simulink model "MMC_21_Level_Rectifier"  (R2023b)
settings: Solver=FixedStepAuto  StartTime=0.0  StopTime=0.5  RelTol=1e-3
libraries: spsSeriesRLCBranchLib x71, spsVoltageMeasurementLib x69, spsUniversalBridgeLib x60, spsCurrentMeasurementLib x8, slpidlib x7, spsRMSLib x3, spsACVoltageSourceLib x3, spsMeanLib x2, simulink x1, spsTHDLib x1, spspowerguiLib x1
(part 3 of 4)

== system MMC_21_Level_Rectifier/三电平级联混合MMC/Subsystem1/Subsystem/混合三电平子模块5 ==
  DRV : Inport
  C0 : spsSeriesRLCBranchLib/Series RLC Branch  LConnTagsString=__new0  RConnTagsString=__new0  BranchType=C  Resistance=0.1  Inductance=0  SetiL0=off  InitialCurrent=0  Capacitance=2e-3  Setx0=on  InitialVoltage=2200  Measurements=None
  C1 : spsSeriesRLCBranchLib/Series RLC Branch  LConnTagsString=__new0  RConnTagsString=__new0  BranchType=C  Resistance=0.1  Inductance=0  SetiL0=off  InitialCurrent=0  Capacitance=2e-3  Setx0=on  InitialVoltage=2200  Measurements=None
  Demux3 : Demux  Outputs=2
  Mux : Mux  Inputs=2
  Universal Bridge1 : spsUniversalBridgeLib/Universal Bridge  Arms=1  SnubberResistance=1e6  SnubberCapacitance=inf  Device=IGBT / Diodes  Ron=1e-3  Lon=0  ForwardVoltages="[  1  1  ]"  ForwardVoltage=0  GTOparameters=[ 10e-6 , 20e-6 ]  IGBTparameters=[ 1e-6 , 2e-6 ]  Measurements=None  Measurements_2=None  converterType=Rectifier
  Universal Bridge2 : spsUniversalBridgeLib/Universal Bridge  Arms=1  SnubberResistance=1e6  SnubberCapacitance=inf  Device=IGBT / Diodes  Ron=1e-3  Lon=0  ForwardVoltages="[  1  1  ]"  ForwardVoltage=0  GTOparameters=[ 10e-6 , 20e-6 ]  IGBTparameters=[ 1e-6 , 2e-6 ]  Measurements=None  Measurements_2=None  converterType=Rectifier
  Vm1 : spsVoltageMeasurementLib/Voltage Measurement  PhasorSimulation=off  OutputType=Complex  PSBequivalent=0
  Vm3 : spsVoltageMeasurementLib/Voltage Measurement  PhasorSimulation=off  OutputType=Complex  PSBequivalent=0
  A : PMIOPort  Side=Left
  B : PMIOPort  Port=2  Side=Left
  Udc : Outport
  wires:
  Mux/1 -> Udc/1
  DRV/1 -> Demux3/1
  Demux3/2 -> Universal Bridge2/1
  Vm1/1 -> Mux/1
  Vm3/1 -> Mux/2
  Demux3/1 -> Universal Bridge1/1
  connections:
  Vm1/LConn2 -- C0/RConn1 -- Universal Bridge1/RConn2 -- Universal Bridge2/LConn1
  Universal Bridge1/LConn1 -- A/RConn1
  Vm3/LConn1 -- C1/LConn1 -- Universal Bridge2/RConn1
  Vm1/LConn1 -- Universal Bridge1/RConn1 -- C0/LConn1
  Universal Bridge2/RConn2 -- C1/RConn1 -- B/RConn1 -- Vm3/LConn2

== system MMC_21_Level_Rectifier/三电平级联混合MMC/Subsystem1/Subsystem1/混合三电平子模块1 ==
  DRV : Inport
  C0 : spsSeriesRLCBranchLib/Series RLC Branch  LConnTagsString=__new0  RConnTagsString=__new0  BranchType=C  Resistance=0.1  Inductance=0  SetiL0=off  InitialCurrent=0  Capacitance=2e-3  Setx0=on  InitialVoltage=2200  Measurements=None
  C1 : spsSeriesRLCBranchLib/Series RLC Branch  LConnTagsString=__new0  RConnTagsString=__new0  BranchType=C  Resistance=0.1  Inductance=0  SetiL0=off  InitialCurrent=0  Capacitance=2e-3  Setx0=on  InitialVoltage=2200  Measurements=None
  Demux3 : Demux  Outputs=2
  Mux : Mux  Inputs=2
  Universal Bridge1 : spsUniversalBridgeLib/Universal Bridge  Arms=1  SnubberResistance=1e6  SnubberCapacitance=inf  Device=IGBT / Diodes  Ron=1e-3  Lon=0  ForwardVoltages="[  1  1  ]"  ForwardVoltage=0  GTOparameters=[ 10e-6 , 20e-6 ]  IGBTparameters=[ 1e-6 , 2e-6 ]  Measurements=None  Measurements_2=None  converterType=Rectifier
  Universal Bridge2 : spsUniversalBridgeLib/Universal Bridge  Arms=1  SnubberResistance=1e6  SnubberCapacitance=inf  Device=IGBT / Diodes  Ron=1e-3  Lon=0  ForwardVoltages="[  1  1  ]"  ForwardVoltage=0  GTOparameters=[ 10e-6 , 20e-6 ]  IGBTparameters=[ 1e-6 , 2e-6 ]  Measurements=None  Measurements_2=None  converterType=Rectifier
  Vm1 : spsVoltageMeasurementLib/Voltage Measurement  PhasorSimulation=off  OutputType=Complex  PSBequivalent=0
  Vm3 : spsVoltageMeasurementLib/Voltage Measurement  PhasorSimulation=off  OutputType=Complex  PSBequivalent=0
  A : PMIOPort  Side=Left
  B : PMIOPort  Port=2  Side=Left
  Udc : Outport
  wires:
  Demux3/1 -> Universal Bridge1/1
  Vm3/1 -> Mux/2
  Vm1/1 -> Mux/1
  Demux3/2 -> Universal Bridge2/1
  DRV/1 -> Demux3/1
  Mux/1 -> Udc/1
  connections:
  Vm3/LConn2 -- B/RConn1 -- C1/RConn1 -- Universal Bridge2/RConn2
  C0/LConn1 -- Universal Bridge1/RConn1 -- Vm1/LConn1
  Universal Bridge2/RConn1 -- C1/LConn1 -- Vm3/LConn1
  Universal Bridge1/LConn1 -- A/RConn1
  Universal Bridge2/LConn1 -- Universal Bridge1/RConn2 -- C0/RConn1 -- Vm1/LConn2

== system MMC_21_Level_Rectifier/三电平级联混合MMC/Subsystem1/Subsystem1/混合三电平子模块2 ==
  DRV : Inport
  C0 : spsSeriesRLCBranchLib/Series RLC Branch  LConnTagsString=__new0  RConnTagsString=__new0  BranchType=C  Resistance=0.1  Inductance=0  SetiL0=off  InitialCurrent=0  Capacitance=2e-3  Setx0=on  InitialVoltage=2200  Measurements=None
  C1 : spsSeriesRLCBranchLib/Series RLC Branch  LConnTagsString=__new0  RConnTagsString=__new0  BranchType=C  Resistance=0.1  Inductance=0  SetiL0=off  InitialCurrent=0  Capacitance=2e-3  Setx0=on  InitialVoltage=2200  Measurements=None
  Demux3 : Demux  Outputs=2
  Mux : Mux  Inputs=2
  Universal Bridge1 : spsUniversalBridgeLib/Universal Bridge  Arms=1  SnubberResistance=1e6  SnubberCapacitance=inf  Device=IGBT / Diodes  Ron=1e-3  Lon=0  ForwardVoltages="[  1  1  ]"  ForwardVoltage=0  GTOparameters=[ 10e-6 , 20e-6 ]  IGBTparameters=[ 1e-6 , 2e-6 ]  Measurements=None  Measurements_2=None  converterType=Rectifier
  Universal Bridge2 : spsUniversalBridgeLib/Universal Bridge  Arms=1  SnubberResistance=1e6  SnubberCapacitance=inf  Device=IGBT / Diodes  Ron=1e-3  Lon=0  ForwardVoltages="[  1  1  ]"  ForwardVoltage=0  GTOparameters=[ 10e-6 , 20e-6 ]  IGBTparameters=[ 1e-6 , 2e-6 ]  Measurements=None  Measurements_2=None  converterType=Rectifier
  Vm1 : spsVoltageMeasurementLib/Voltage Measurement  PhasorSimulation=off  OutputType=Complex  PSBequivalent=0
  Vm3 : spsVoltageMeasurementLib/Voltage Measurement  PhasorSimulation=off  OutputType=Complex  PSBequivalent=0
  A : PMIOPort  Side=Left
  B : PMIOPort  Port=2  Side=Left
  Udc : Outport
  wires:
  Mux/1 -> Udc/1
  DRV/1 -> Demux3/1
  Demux3/2 -> Universal Bridge2/1
  Vm1/1 -> Mux/1
  Vm3/1 -> Mux/2
  Demux3/1 -> Universal Bridge1/1
  connections:
  Vm1/LConn2 -- C0/RConn1 -- Universal Bridge1/RConn2 -- Universal Bridge2/LConn1
  Universal Bridge1/LConn1 -- A/RConn1
  Vm3/LConn1 -- C1/LConn1 -- Universal Bridge2/RConn1
  Vm1/LConn1 -- Universal Bridge1/RConn1 -- C0/LConn1
  Universal Bridge2/RConn2 -- C1/RConn1 -- B/RConn1 -- Vm3/LConn2

== system MMC_21_Level_Rectifier/三电平级联混合MMC/Subsystem1/Subsystem1/混合三电平子模块3 ==
  DRV : Inport
  C0 : spsSeriesRLCBranchLib/Series RLC Branch  LConnTagsString=__new0  RConnTagsString=__new0  BranchType=C  Resistance=0.1  Inductance=0  SetiL0=off  InitialCurrent=0  Capacitance=2e-3  Setx0=on  InitialVoltage=2200  Measurements=None
  C1 : spsSeriesRLCBranchLib/Series RLC Branch  LConnTagsString=__new0  RConnTagsString=__new0  BranchType=C  Resistance=0.1  Inductance=0  SetiL0=off  InitialCurrent=0  Capacitance=2e-3  Setx0=on  InitialVoltage=2200  Measurements=None
  Demux3 : Demux  Outputs=2
  Mux : Mux  Inputs=2
  Universal Bridge1 : spsUniversalBridgeLib/Universal Bridge  Arms=1  SnubberResistance=1e6  SnubberCapacitance=inf  Device=IGBT / Diodes  Ron=1e-3  Lon=0  ForwardVoltages="[  1  1  ]"  ForwardVoltage=0  GTOparameters=[ 10e-6 , 20e-6 ]  IGBTparameters=[ 1e-6 , 2e-6 ]  Measurements=None  Measurements_2=None  converterType=Rectifier
  Universal Bridge2 : spsUniversalBridgeLib/Universal Bridge  Arms=1  SnubberResistance=1e6  SnubberCapacitance=inf  Device=IGBT / Diodes  Ron=1e-3  Lon=0  ForwardVoltages="[  1  1  ]"  ForwardVoltage=0  GTOparameters=[ 10e-6 , 20e-6 ]  IGBTparameters=[ 1e-6 , 2e-6 ]  Measurements=None  Measurements_2=None  converterType=Rectifier
  Vm1 : spsVoltageMeasurementLib/Voltage Measurement  PhasorSimulation=off  OutputType=Complex  PSBequivalent=0
  Vm3 : spsVoltageMeasurementLib/Voltage Measurement  PhasorSimulation=off  OutputType=Complex  PSBequivalent=0
  A : PMIOPort  Side=Left
  B : PMIOPort  Port=2  Side=Left
  Udc : Outport
  wires:
  Demux3/1 -> Universal Bridge1/1
  Vm3/1 -> Mux/2
  Vm1/1 -> Mux/1
  Demux3/2 -> Universal Bridge2/1
  DRV/1 -> Demux3/1
  Mux/1 -> Udc/1
  connections:
  Vm3/LConn2 -- B/RConn1 -- C1/RConn1 -- Universal Bridge2/RConn2
  C0/LConn1 -- Universal Bridge1/RConn1 -- Vm1/LConn1
  Universal Bridge2/RConn1 -- C1/LConn1 -- Vm3/LConn1
  Universal Bridge1/LConn1 -- A/RConn1
  Universal Bridge2/LConn1 -- Universal Bridge1/RConn2 -- C0/RConn1 -- Vm1/LConn2

== system MMC_21_Level_Rectifier/三电平级联混合MMC/Subsystem1/Subsystem1/混合三电平子模块4 ==
  DRV : Inport
  C0 : spsSeriesRLCBranchLib/Series RLC Branch  LConnTagsString=__new0  RConnTagsString=__new0  BranchType=C  Resistance=0.1  Inductance=0  SetiL0=off  InitialCurrent=0  Capacitance=2e-3  Setx0=on  InitialVoltage=2200  Measurements=None
  C1 : spsSeriesRLCBranchLib/Series RLC Branch  LConnTagsString=__new0  RConnTagsString=__new0  BranchType=C  Resistance=0.1  Inductance=0  SetiL0=off  InitialCurrent=0  Capacitance=2e-3  Setx0=on  InitialVoltage=2200  Measurements=None
  Demux3 : Demux  Outputs=2
  Mux : Mux  Inputs=2
  Universal Bridge1 : spsUniversalBridgeLib/Universal Bridge  Arms=1  SnubberResistance=1e6  SnubberCapacitance=inf  Device=IGBT / Diodes  Ron=1e-3  Lon=0  ForwardVoltages="[  1  1  ]"  ForwardVoltage=0  GTOparameters=[ 10e-6 , 20e-6 ]  IGBTparameters=[ 1e-6 , 2e-6 ]  Measurements=None  Measurements_2=None  converterType=Rectifier
  Universal Bridge2 : spsUniversalBridgeLib/Universal Bridge  Arms=1  SnubberResistance=1e6  SnubberCapacitance=inf  Device=IGBT / Diodes  Ron=1e-3  Lon=0  ForwardVoltages="[  1  1  ]"  ForwardVoltage=0  GTOparameters=[ 10e-6 , 20e-6 ]  IGBTparameters=[ 1e-6 , 2e-6 ]  Measurements=None  Measurements_2=None  converterType=Rectifier
  Vm1 : spsVoltageMeasurementLib/Voltage Measurement  PhasorSimulation=off  OutputType=Complex  PSBequivalent=0
  Vm3 : spsVoltageMeasurementLib/Voltage Measurement  PhasorSimulation=off  OutputType=Complex  PSBequivalent=0
  A : PMIOPort  Side=Left
  B : PMIOPort  Port=2  Side=Left
  Udc : Outport
  wires:
  Mux/1 -> Udc/1
  DRV/1 -> Demux3/1
  Demux3/2 -> Universal Bridge2/1
  Vm1/1 -> Mux/1
  Vm3/1 -> Mux/2
  Demux3/1 -> Universal Bridge1/1
  connections:
  Vm1/LConn2 -- C0/RConn1 -- Universal Bridge1/RConn2 -- Universal Bridge2/LConn1
  Universal Bridge1/LConn1 -- A/RConn1
  Vm3/LConn1 -- C1/LConn1 -- Universal Bridge2/RConn1
  Vm1/LConn1 -- Universal Bridge1/RConn1 -- C0/LConn1
  Universal Bridge2/RConn2 -- C1/RConn1 -- B/RConn1 -- Vm3/LConn2

== system MMC_21_Level_Rectifier/三电平级联混合MMC/Subsystem1/Subsystem1/混合三电平子模块5 ==
  DRV : Inport
  C0 : spsSeriesRLCBranchLib/Series RLC Branch  LConnTagsString=__new0  RConnTagsString=__new0  BranchType=C  Resistance=0.1  Inductance=0  SetiL0=off  InitialCurrent=0  Capacitance=2e-3  Setx0=on  InitialVoltage=2200  Measurements=None
  C1 : spsSeriesRLCBranchLib/Series RLC Branch  LConnTagsString=__new0  RConnTagsString=__new0  BranchType=C  Resistance=0.1  Inductance=0  SetiL0=off  InitialCurrent=0  Capacitance=2e-3  Setx0=on  InitialVoltage=2200  Measurements=None
  Demux3 : Demux  Outputs=2
  Mux : Mux  Inputs=2
  Universal Bridge1 : spsUniversalBridgeLib/Universal Bridge  Arms=1  SnubberResistance=1e6  SnubberCapacitance=inf  Device=IGBT / Diodes  Ron=1e-3  Lon=0  ForwardVoltages="[  1  1  ]"  ForwardVoltage=0  GTOparameters=[ 10e-6 , 20e-6 ]  IGBTparameters=[ 1e-6 , 2e-6 ]  Measurements=None  Measurements_2=None  converterType=Rectifier
  Universal Bridge2 : spsUniversalBridgeLib/Universal Bridge  Arms=1  SnubberResistance=1e6  SnubberCapacitance=inf  Device=IGBT / Diodes  Ron=1e-3  Lon=0  ForwardVoltages="[  1  1  ]"  ForwardVoltage=0  GTOparameters=[ 10e-6 , 20e-6 ]  IGBTparameters=[ 1e-6 , 2e-6 ]  Measurements=None  Measurements_2=None  converterType=Rectifier
  Vm1 : spsVoltageMeasurementLib/Voltage Measurement  PhasorSimulation=off  OutputType=Complex  PSBequivalent=0
  Vm3 : spsVoltageMeasurementLib/Voltage Measurement  PhasorSimulation=off  OutputType=Complex  PSBequivalent=0
  A : PMIOPort  Side=Left
  B : PMIOPort  Port=2  Side=Left
  Udc : Outport
  wires:
  Demux3/1 -> Universal Bridge1/1
  Vm3/1 -> Mux/2
  Vm1/1 -> Mux/1
  Demux3/2 -> Universal Bridge2/1
  DRV/1 -> Demux3/1
  Mux/1 -> Udc/1
  connections:
  Vm3/LConn2 -- B/RConn1 -- C1/RConn1 -- Universal Bridge2/RConn2
  C0/LConn1 -- Universal Bridge1/RConn1 -- Vm1/LConn1
  Universal Bridge2/RConn1 -- C1/LConn1 -- Vm3/LConn1
  Universal Bridge1/LConn1 -- A/RConn1
  Universal Bridge2/LConn1 -- Universal Bridge1/RConn2 -- C0/RConn1 -- Vm1/LConn2

== system MMC_21_Level_Rectifier/三电平级联混合MMC/Subsystem2/Subsystem/混合三电平子模块1 ==
  DRV : Inport
  C0 : spsSeriesRLCBranchLib/Series RLC Branch  LConnTagsString=__new0  RConnTagsString=__new0  BranchType=C  Resistance=0.1  Inductance=0  SetiL0=off  InitialCurrent=0  Capacitance=2e-3  Setx0=on  InitialVoltage=2200  Measurements=None
  C1 : spsSeriesRLCBranchLib/Series RLC Branch  LConnTagsString=__new0  RConnTagsString=__new0  BranchType=C  Resistance=0.1  Inductance=0  SetiL0=off  InitialCurrent=0  Capacitance=2e-3  Setx0=on  InitialVoltage=2200  Measurements=None
  Demux3 : Demux  Outputs=2
  Mux : Mux  Inputs=2
  Universal Bridge1 : spsUniversalBridgeLib/Universal Bridge  Arms=1  SnubberResistance=1e6  SnubberCapacitance=inf  Device=IGBT / Diodes  Ron=1e-3  Lon=0  ForwardVoltages="[  1  1  ]"  ForwardVoltage=0  GTOparameters=[ 10e-6 , 20e-6 ]  IGBTparameters=[ 1e-6 , 2e-6 ]  Measurements=None  Measurements_2=None  converterType=Rectifier
  Universal Bridge2 : spsUniversalBridgeLib/Universal Bridge  Arms=1  SnubberResistance=1e6  SnubberCapacitance=inf  Device=IGBT / Diodes  Ron=1e-3  Lon=0  ForwardVoltages="[  1  1  ]"  ForwardVoltage=0  GTOparameters=[ 10e-6 , 20e-6 ]  IGBTparameters=[ 1e-6 , 2e-6 ]  Measurements=None  Measurements_2=None  converterType=Rectifier
  Vm1 : spsVoltageMeasurementLib/Voltage Measurement  PhasorSimulation=off  OutputType=Complex  PSBequivalent=0
  Vm3 : spsVoltageMeasurementLib/Voltage Measurement  PhasorSimulation=off  OutputType=Complex  PSBequivalent=0
  A : PMIOPort  Side=Left
  B : PMIOPort  Port=2  Side=Left
  Udc : Outport
  wires:
  Demux3/1 -> Universal Bridge1/1
  Vm3/1 -> Mux/2
  Vm1/1 -> Mux/1
  Demux3/2 -> Universal Bridge2/1
  DRV/1 -> Demux3/1
  Mux/1 -> Udc/1
  connections:
  C1/RConn1 -- Universal Bridge2/RConn2 -- Vm3/LConn2 -- B/RConn1
  C0/LConn1 -- Universal Bridge1/RConn1 -- Vm1/LConn1
  C1/LConn1 -- Vm3/LConn1 -- Universal Bridge2/RConn1
  Universal Bridge1/LConn1 -- A/RConn1
  C0/RConn1 -- Universal Bridge2/LConn1 -- Vm1/LConn2 -- Universal Bridge1/RConn2

== system MMC_21_Level_Rectifier/三电平级联混合MMC/Subsystem2/Subsystem/混合三电平子模块2 ==
  DRV : Inport
  C0 : spsSeriesRLCBranchLib/Series RLC Branch  LConnTagsString=__new0  RConnTagsString=__new0  BranchType=C  Resistance=0.1  Inductance=0  SetiL0=off  InitialCurrent=0  Capacitance=2e-3  Setx0=on  InitialVoltage=2200  Measurements=None
  C1 : spsSeriesRLCBranchLib/Series RLC Branch  LConnTagsString=__new0  RConnTagsString=__new0  BranchType=C  Resistance=0.1  Inductance=0  SetiL0=off  InitialCurrent=0  Capacitance=2e-3  Setx0=on  InitialVoltage=2200  Measurements=None
  Demux3 : Demux  Outputs=2
  Mux : Mux  Inputs=2
  Universal Bridge1 : spsUniversalBridgeLib/Universal Bridge  Arms=1  SnubberResistance=1e6  SnubberCapacitance=inf  Device=IGBT / Diodes  Ron=1e-3  Lon=0  ForwardVoltages="[  1  1  ]"  ForwardVoltage=0  GTOparameters=[ 10e-6 , 20e-6 ]  IGBTparameters=[ 1e-6 , 2e-6 ]  Measurements=None  Measurements_2=None  converterType=Rectifier
  Universal Bridge2 : spsUniversalBridgeLib/Universal Bridge  Arms=1  SnubberResistance=1e6  SnubberCapacitance=inf  Device=IGBT / Diodes  Ron=1e-3  Lon=0  ForwardVoltages="[  1  1  ]"  ForwardVoltage=0  GTOparameters=[ 10e-6 , 20e-6 ]  IGBTparameters=[ 1e-6 , 2e-6 ]  Measurements=None  Measurements_2=None  converterType=Rectifier
  Vm1 : spsVoltageMeasurementLib/Voltage Measurement  PhasorSimulation=off  OutputType=Complex  PSBequivalent=0
  Vm3 : spsVoltageMeasurementLib/Voltage Measurement  PhasorSimulation=off  OutputType=Complex  PSBequivalent=0
  A : PMIOPort  Side=Left
  B : PMIOPort  Port=2  Side=Left
  Udc : Outport
  wires:
  Mux/1 -> Udc/1
  DRV/1 -> Demux3/1
  Demux3/2 -> Universal Bridge2/1
  Vm1/1 -> Mux/1
  Vm3/1 -> Mux/2
  Demux3/1 -> Universal Bridge1/1
  connections:
  Vm1/LConn2 -- C0/RConn1 -- Universal Bridge1/RConn2 -- Universal Bridge2/LConn1
  Universal Bridge1/LConn1 -- A/RConn1
  Vm3/LConn1 -- C1/LConn1 -- Universal Bridge2/RConn1
  Vm1/LConn1 -- Universal Bridge1/RConn1 -- C0/LConn1
  Universal Bridge2/RConn2 -- C1/RConn1 -- B/RConn1 -- Vm3/LConn2

== system MMC_21_Level_Rectifier/三电平级联混合MMC/Subsystem2/Subsystem/混合三电平子模块3 ==
  DRV : Inport
  C0 : spsSeriesRLCBranchLib/Series RLC Branch  LConnTagsString=__new0  RConnTagsString=__new0  BranchType=C  Resistance=0.1  Inductance=0  SetiL0=off  InitialCurrent=0  Capacitance=2e-3  Setx0=on  InitialVoltage=2200  Measurements=None
  C1 : spsSeriesRLCBranchLib/Series RLC Branch  LConnTagsString=__new0  RConnTagsString=__new0  BranchType=C  Resistance=0.1  Inductance=0  SetiL0=off  InitialCurrent=0  Capacitance=2e-3  Setx0=on  InitialVoltage=2200  Measurements=None
  Demux3 : Demux  Outputs=2
  Mux : Mux  Inputs=2
  Universal Bridge1 : spsUniversalBridgeLib/Universal Bridge  Arms=1  SnubberResistance=1e6  SnubberCapacitance=inf  Device=IGBT / Diodes  Ron=1e-3  Lon=0  ForwardVoltages="[  1  1  ]"  ForwardVoltage=0  GTOparameters=[ 10e-6 , 20e-6 ]  IGBTparameters=[ 1e-6 , 2e-6 ]  Measurements=None  Measurements_2=None  converterType=Rectifier
  Universal Bridge2 : spsUniversalBridgeLib/Universal Bridge  Arms=1  SnubberResistance=1e6  SnubberCapacitance=inf  Device=IGBT / Diodes  Ron=1e-3  Lon=0  ForwardVoltages="[  1  1  ]"  ForwardVoltage=0  GTOparameters=[ 10e-6 , 20e-6 ]  IGBTparameters=[ 1e-6 , 2e-6 ]  Measurements=None  Measurements_2=None  converterType=Rectifier
  Vm1 : spsVoltageMeasurementLib/Voltage Measurement  PhasorSimulation=off  OutputType=Complex  PSBequivalent=0
  Vm3 : spsVoltageMeasurementLib/Voltage Measurement  PhasorSimulation=off  OutputType=Complex  PSBequivalent=0
  A : PMIOPort  Side=Left
  B : PMIOPort  Port=2  Side=Left
  Udc : Outport
  wires:
  Demux3/1 -> Universal Bridge1/1
  Vm3/1 -> Mux/2
  Vm1/1 -> Mux/1
  Demux3/2 -> Universal Bridge2/1
  DRV/1 -> Demux3/1
  Mux/1 -> Udc/1
  connections:
  Vm3/LConn2 -- B/RConn1 -- C1/RConn1 -- Universal Bridge2/RConn2
  C0/LConn1 -- Universal Bridge1/RConn1 -- Vm1/LConn1
  Universal Bridge2/RConn1 -- C1/LConn1 -- Vm3/LConn1
  Universal Bridge1/LConn1 -- A/RConn1
  Universal Bridge2/LConn1 -- Universal Bridge1/RConn2 -- C0/RConn1 -- Vm1/LConn2

== system MMC_21_Level_Rectifier/三电平级联混合MMC/Subsystem2/Subsystem/混合三电平子模块4 ==
  DRV : Inport
  C0 : spsSeriesRLCBranchLib/Series RLC Branch  LConnTagsString=__new0  RConnTagsString=__new0  BranchType=C  Resistance=0.1  Inductance=0  SetiL0=off  InitialCurrent=0  Capacitance=2e-3  Setx0=on  InitialVoltage=2200  Measurements=None
  C1 : spsSeriesRLCBranchLib/Series RLC Branch  LConnTagsString=__new0  RConnTagsString=__new0  BranchType=C  Resistance=0.1  Inductance=0  SetiL0=off  InitialCurrent=0  Capacitance=2e-3  Setx0=on  InitialVoltage=2200  Measurements=None
  Demux3 : Demux  Outputs=2
  Mux : Mux  Inputs=2
  Universal Bridge1 : spsUniversalBridgeLib/Universal Bridge  Arms=1  SnubberResistance=1e6  SnubberCapacitance=inf  Device=IGBT / Diodes  Ron=1e-3  Lon=0  ForwardVoltages="[  1  1  ]"  ForwardVoltage=0  GTOparameters=[ 10e-6 , 20e-6 ]  IGBTparameters=[ 1e-6 , 2e-6 ]  Measurements=None  Measurements_2=None  converterType=Rectifier
  Universal Bridge2 : spsUniversalBridgeLib/Universal Bridge  Arms=1  SnubberResistance=1e6  SnubberCapacitance=inf  Device=IGBT / Diodes  Ron=1e-3  Lon=0  ForwardVoltages="[  1  1  ]"  ForwardVoltage=0  GTOparameters=[ 10e-6 , 20e-6 ]  IGBTparameters=[ 1e-6 , 2e-6 ]  Measurements=None  Measurements_2=None  converterType=Rectifier
  Vm1 : spsVoltageMeasurementLib/Voltage Measurement  PhasorSimulation=off  OutputType=Complex  PSBequivalent=0
  Vm3 : spsVoltageMeasurementLib/Voltage Measurement  PhasorSimulation=off  OutputType=Complex  PSBequivalent=0
  A : PMIOPort  Side=Left
  B : PMIOPort  Port=2  Side=Left
  Udc : Outport
  wires:
  Mux/1 -> Udc/1
  DRV/1 -> Demux3/1
  Demux3/2 -> Universal Bridge2/1
  Vm1/1 -> Mux/1
  Vm3/1 -> Mux/2
  Demux3/1 -> Universal Bridge1/1
  connections:
  Vm1/LConn2 -- C0/RConn1 -- Universal Bridge1/RConn2 -- Universal Bridge2/LConn1
  Universal Bridge1/LConn1 -- A/RConn1
  Vm3/LConn1 -- C1/LConn1 -- Universal Bridge2/RConn1
  Vm1/LConn1 -- Universal Bridge1/RConn1 -- C0/LConn1
  Universal Bridge2/RConn2 -- C1/RConn1 -- B/RConn1 -- Vm3/LConn2

== system MMC_21_Level_Rectifier/三电平级联混合MMC/Subsystem2/Subsystem/混合三电平子模块5 ==
  DRV : Inport
  C0 : spsSeriesRLCBranchLib/Series RLC Branch  LConnTagsString=__new0  RConnTagsString=__new0  BranchType=C  Resistance=0.1  Inductance=0  SetiL0=off  InitialCurrent=0  Capacitance=2e-3  Setx0=on  InitialVoltage=2200  Measurements=None
  C1 : spsSeriesRLCBranchLib/Series RLC Branch  LConnTagsString=__new0  RConnTagsString=__new0  BranchType=C  Resistance=0.1  Inductance=0  SetiL0=off  InitialCurrent=0  Capacitance=2e-3  Setx0=on  InitialVoltage=2200  Measurements=None
  Demux3 : Demux  Outputs=2
  Mux : Mux  Inputs=2
  Universal Bridge1 : spsUniversalBridgeLib/Universal Bridge  Arms=1  SnubberResistance=1e6  SnubberCapacitance=inf  Device=IGBT / Diodes  Ron=1e-3  Lon=0  ForwardVoltages="[  1  1  ]"  ForwardVoltage=0  GTOparameters=[ 10e-6 , 20e-6 ]  IGBTparameters=[ 1e-6 , 2e-6 ]  Measurements=None  Measurements_2=None  converterType=Rectifier
  Universal Bridge2 : spsUniversalBridgeLib/Universal Bridge  Arms=1  SnubberResistance=1e6  SnubberCapacitance=inf  Device=IGBT / Diodes  Ron=1e-3  Lon=0  ForwardVoltages="[  1  1  ]"  ForwardVoltage=0  GTOparameters=[ 10e-6 , 20e-6 ]  IGBTparameters=[ 1e-6 , 2e-6 ]  Measurements=None  Measurements_2=None  converterType=Rectifier
  Vm1 : spsVoltageMeasurementLib/Voltage Measurement  PhasorSimulation=off  OutputType=Complex  PSBequivalent=0
  Vm3 : spsVoltageMeasurementLib/Voltage Measurement  PhasorSimulation=off  OutputType=Complex  PSBequivalent=0
  A : PMIOPort  Side=Left
  B : PMIOPort  Port=2  Side=Left
  Udc : Outport
  wires:
  Demux3/1 -> Universal Bridge1/1
  Vm3/1 -> Mux/2
  Vm1/1 -> Mux/1
  Demux3/2 -> Universal Bridge2/1
  DRV/1 -> Demux3/1
  Mux/1 -> Udc/1
  connections:
  Vm3/LConn2 -- B/RConn1 -- C1/RConn1 -- Universal Bridge2/RConn2
  C0/LConn1 -- Universal Bridge1/RConn1 -- Vm1/LConn1
  Universal Bridge2/RConn1 -- C1/LConn1 -- Vm3/LConn1
  Universal Bridge1/LConn1 -- A/RConn1
  Universal Bridge2/LConn1 -- Universal Bridge1/RConn2 -- C0/RConn1 -- Vm1/LConn2

== system MMC_21_Level_Rectifier/三电平级联混合MMC/Subsystem2/Subsystem1/混合三电平子模块1 ==
  DRV : Inport
  C0 : spsSeriesRLCBranchLib/Series RLC Branch  LConnTagsString=__new0  RConnTagsString=__new0  BranchType=C  Resistance=0.1  Inductance=0  SetiL0=off  InitialCurrent=0  Capacitance=2e-3  Setx0=on  InitialVoltage=2200  Measurements=None
  C1 : spsSeriesRLCBranchLib/Series RLC Branch  LConnTagsString=__new0  RConnTagsString=__new0  BranchType=C  Resistance=0.1  Inductance=0  SetiL0=off  InitialCurrent=0  Capacitance=2e-3  Setx0=on  InitialVoltage=2200  Measurements=None
  Demux3 : Demux  Outputs=2
  Mux : Mux  Inputs=2
  Universal Bridge1 : spsUniversalBridgeLib/Universal Bridge  Arms=1  SnubberResistance=1e6  SnubberCapacitance=inf  Device=IGBT / Diodes  Ron=1e-3  Lon=0  ForwardVoltages="[  1  1  ]"  ForwardVoltage=0  GTOparameters=[ 10e-6 , 20e-6 ]  IGBTparameters=[ 1e-6 , 2e-6 ]  Measurements=None  Measurements_2=None  converterType=Rectifier
  Universal Bridge2 : spsUniversalBridgeLib/Universal Bridge  Arms=1  SnubberResistance=1e6  SnubberCapacitance=inf  Device=IGBT / Diodes  Ron=1e-3  Lon=0  ForwardVoltages="[  1  1  ]"  ForwardVoltage=0  GTOparameters=[ 10e-6 , 20e-6 ]  IGBTparameters=[ 1e-6 , 2e-6 ]  Measurements=None  Measurements_2=None  converterType=Rectifier
  Vm1 : spsVoltageMeasurementLib/Voltage Measurement  PhasorSimulation=off  OutputType=Complex  PSBequivalent=0
  Vm3 : spsVoltageMeasurementLib/Voltage Measurement  PhasorSimulation=off  OutputType=Complex  PSBequivalent=0
  A : PMIOPort  Side=Left
  B : PMIOPort  Port=2  Side=Left
  Udc : Outport
  wires:
  Mux/1 -> Udc/1
  DRV/1 -> Demux3/1
  Demux3/2 -> Universal Bridge2/1
  Vm1/1 -> Mux/1
  Vm3/1 -> Mux/2
  Demux3/1 -> Universal Bridge1/1
  connections:
  Vm1/LConn2 -- C0/RConn1 -- Universal Bridge1/RConn2 -- Universal Bridge2/LConn1
  Universal Bridge1/LConn1 -- A/RConn1
  Vm3/LConn1 -- C1/LConn1 -- Universal Bridge2/RConn1
  Vm1/LConn1 -- Universal Bridge1/RConn1 -- C0/LConn1
  Universal Bridge2/RConn2 -- C1/RConn1 -- B/RConn1 -- Vm3/LConn2

== system MMC_21_Level_Rectifier/三电平级联混合MMC/Subsystem2/Subsystem1/混合三电平子模块2 ==
  DRV : Inport
  C0 : spsSeriesRLCBranchLib/Series RLC Branch  LConnTagsString=__new0  RConnTagsString=__new0  BranchType=C  Resistance=0.1  Inductance=0  SetiL0=off  InitialCurrent=0  Capacitance=2e-3  Setx0=on  InitialVoltage=2200  Measurements=None
  C1 : spsSeriesRLCBranchLib/Series RLC Branch  LConnTagsString=__new0  RConnTagsString=__new0  BranchType=C  Resistance=0.1  Inductance=0  SetiL0=off  InitialCurrent=0  Capacitance=2e-3  Setx0=on  InitialVoltage=2200  Measurements=None
  Demux3 : Demux  Outputs=2
  Mux : Mux  Inputs=2
  Universal Bridge1 : spsUniversalBridgeLib/Universal Bridge  Arms=1  SnubberResistance=1e6  SnubberCapacitance=inf  Device=IGBT / Diodes  Ron=1e-3  Lon=0  ForwardVoltages="[  1  1  ]"  ForwardVoltage=0  GTOparameters=[ 10e-6 , 20e-6 ]  IGBTparameters=[ 1e-6 , 2e-6 ]  Measurements=None  Measurements_2=None  converterType=Rectifier
  Universal Bridge2 : spsUniversalBridgeLib/Universal Bridge  Arms=1  SnubberResistance=1e6  SnubberCapacitance=inf  Device=IGBT / Diodes  Ron=1e-3  Lon=0  ForwardVoltages="[  1  1  ]"  ForwardVoltage=0  GTOparameters=[ 10e-6 , 20e-6 ]  IGBTparameters=[ 1e-6 , 2e-6 ]  Measurements=None  Measurements_2=None  converterType=Rectifier
  Vm1 : spsVoltageMeasurementLib/Voltage Measurement  PhasorSimulation=off  OutputType=Complex  PSBequivalent=0
  Vm3 : spsVoltageMeasurementLib/Voltage Measurement  PhasorSimulation=off  OutputType=Complex  PSBequivalent=0
  A : PMIOPort  Side=Left
  B : PMIOPort  Port=2  Side=Left
  Udc : Outport
  wires:
  Demux3/1 -> Universal Bridge1/1
  Vm3/1 -> Mux/2
  Vm1/1 -> Mux/1
  Demux3/2 -> Universal Bridge2/1
  DRV/1 -> Demux3/1
  Mux/1 -> Udc/1
  connections:
  Vm3/LConn2 -- B/RConn1 -- C1/RConn1 -- Universal Bridge2/RConn2
  C0/LConn1 -- Universal Bridge1/RConn1 -- Vm1/LConn1
  Universal Bridge2/RConn1 -- C1/LConn1 -- Vm3/LConn1
  Universal Bridge1/LConn1 -- A/RConn1
  Universal Bridge2/LConn1 -- Universal Bridge1/RConn2 -- C0/RConn1 -- Vm1/LConn2

== system MMC_21_Level_Rectifier/三电平级联混合MMC/Subsystem2/Subsystem1/混合三电平子模块3 ==
  DRV : Inport
  C0 : spsSeriesRLCBranchLib/Series RLC Branch  LConnTagsString=__new0  RConnTagsString=__new0  BranchType=C  Resistance=0.1  Inductance=0  SetiL0=off  InitialCurrent=0  Capacitance=2e-3  Setx0=on  InitialVoltage=2200  Measurements=None
  C1 : spsSeriesRLCBranchLib/Series RLC Branch  LConnTagsString=__new0  RConnTagsString=__new0  BranchType=C  Resistance=0.1  Inductance=0  SetiL0=off  InitialCurrent=0  Capacitance=2e-3  Setx0=on  InitialVoltage=2200  Measurements=None
  Demux3 : Demux  Outputs=2
  Mux : Mux  Inputs=2
  Universal Bridge1 : spsUniversalBridgeLib/Universal Bridge  Arms=1  SnubberResistance=1e6  SnubberCapacitance=inf  Device=IGBT / Diodes  Ron=1e-3  Lon=0  ForwardVoltages="[  1  1  ]"  ForwardVoltage=0  GTOparameters=[ 10e-6 , 20e-6 ]  IGBTparameters=[ 1e-6 , 2e-6 ]  Measurements=None  Measurements_2=None  converterType=Rectifier
  Universal Bridge2 : spsUniversalBridgeLib/Universal Bridge  Arms=1  SnubberResistance=1e6  SnubberCapacitance=inf  Device=IGBT / Diodes  Ron=1e-3  Lon=0  ForwardVoltages="[  1  1  ]"  ForwardVoltage=0  GTOparameters=[ 10e-6 , 20e-6 ]  IGBTparameters=[ 1e-6 , 2e-6 ]  Measurements=None  Measurements_2=None  converterType=Rectifier
  Vm1 : spsVoltageMeasurementLib/Voltage Measurement  PhasorSimulation=off  OutputType=Complex  PSBequivalent=0
  Vm3 : spsVoltageMeasurementLib/Voltage Measurement  PhasorSimulation=off  OutputType=Complex  PSBequivalent=0
  A : PMIOPort  Side=Left
  B : PMIOPort  Port=2  Side=Left
  Udc : Outport
  wires:
  Mux/1 -> Udc/1
  DRV/1 -> Demux3/1
  Demux3/2 -> Universal Bridge2/1
  Vm1/1 -> Mux/1
  Vm3/1 -> Mux/2
  Demux3/1 -> Universal Bridge1/1
  connections:
  Vm1/LConn2 -- C0/RConn1 -- Universal Bridge1/RConn2 -- Universal Bridge2/LConn1
  Universal Bridge1/LConn1 -- A/RConn1
  Vm3/LConn1 -- C1/LConn1 -- Universal Bridge2/RConn1
  Vm1/LConn1 -- Universal Bridge1/RConn1 -- C0/LConn1
  Universal Bridge2/RConn2 -- C1/RConn1 -- B/RConn1 -- Vm3/LConn2

== system MMC_21_Level_Rectifier/三电平级联混合MMC/Subsystem2/Subsystem1/混合三电平子模块4 ==
  DRV : Inport
  C0 : spsSeriesRLCBranchLib/Series RLC Branch  LConnTagsString=__new0  RConnTagsString=__new0  BranchType=C  Resistance=0.1  Inductance=0  SetiL0=off  InitialCurrent=0  Capacitance=2e-3  Setx0=on  InitialVoltage=2200  Measurements=None
  C1 : spsSeriesRLCBranchLib/Series RLC Branch  LConnTagsString=__new0  RConnTagsString=__new0  BranchType=C  Resistance=0.1  Inductance=0  SetiL0=off  InitialCurrent=0  Capacitance=2e-3  Setx0=on  InitialVoltage=2200  Measurements=None
  Demux3 : Demux  Outputs=2
  Mux : Mux  Inputs=2
  Universal Bridge1 : spsUniversalBridgeLib/Universal Bridge  Arms=1  SnubberResistance=1e6  SnubberCapacitance=inf  Device=IGBT / Diodes  Ron=1e-3  Lon=0  ForwardVoltages="[  1  1  ]"  ForwardVoltage=0  GTOparameters=[ 10e-6 , 20e-6 ]  IGBTparameters=[ 1e-6 , 2e-6 ]  Measurements=None  Measurements_2=None  converterType=Rectifier
  Universal Bridge2 : spsUniversalBridgeLib/Universal Bridge  Arms=1  SnubberResistance=1e6  SnubberCapacitance=inf  Device=IGBT / Diodes  Ron=1e-3  Lon=0  ForwardVoltages="[  1  1  ]"  ForwardVoltage=0  GTOparameters=[ 10e-6 , 20e-6 ]  IGBTparameters=[ 1e-6 , 2e-6 ]  Measurements=None  Measurements_2=None  converterType=Rectifier
  Vm1 : spsVoltageMeasurementLib/Voltage Measurement  PhasorSimulation=off  OutputType=Complex  PSBequivalent=0
  Vm3 : spsVoltageMeasurementLib/Voltage Measurement  PhasorSimulation=off  OutputType=Complex  PSBequivalent=0
  A : PMIOPort  Side=Left
  B : PMIOPort  Port=2  Side=Left
  Udc : Outport
  wires:
  Demux3/1 -> Universal Bridge1/1
  Vm3/1 -> Mux/2
  Vm1/1 -> Mux/1
  Demux3/2 -> Universal Bridge2/1
  DRV/1 -> Demux3/1
  Mux/1 -> Udc/1
  connections:
  Vm3/LConn2 -- B/RConn1 -- C1/RConn1 -- Universal Bridge2/RConn2
  C0/LConn1 -- Universal Bridge1/RConn1 -- Vm1/LConn1
  Universal Bridge2/RConn1 -- C1/LConn1 -- Vm3/LConn1
  Universal Bridge1/LConn1 -- A/RConn1
  Universal Bridge2/LConn1 -- Universal Bridge1/RConn2 -- C0/RConn1 -- Vm1/LConn2

== system MMC_21_Level_Rectifier/三电平级联混合MMC/Subsystem2/Subsystem1/混合三电平子模块5 ==
  DRV : Inport
  C0 : spsSeriesRLCBranchLib/Series RLC Branch  LConnTagsString=__new0  RConnTagsString=__new0  BranchType=C  Resistance=0.1  Inductance=0  SetiL0=off  InitialCurrent=0  Capacitance=2e-3  Setx0=on  InitialVoltage=2200  Measurements=None
  C1 : spsSeriesRLCBranchLib/Series RLC Branch  LConnTagsString=__new0  RConnTagsString=__new0  BranchType=C  Resistance=0.1  Inductance=0  SetiL0=off  InitialCurrent=0  Capacitance=2e-3  Setx0=on  InitialVoltage=2200  Measurements=None
  Demux3 : Demux  Outputs=2
  Mux : Mux  Inputs=2
  Universal Bridge1 : spsUniversalBridgeLib/Universal Bridge  Arms=1  SnubberResistance=1e6  SnubberCapacitance=inf  Device=IGBT / Diodes  Ron=1e-3  Lon=0  ForwardVoltages="[  1  1  ]"  ForwardVoltage=0  GTOparameters=[ 10e-6 , 20e-6 ]  IGBTparameters=[ 1e-6 , 2e-6 ]  Measurements=None  Measurements_2=None  converterType=Rectifier
  Universal Bridge2 : spsUniversalBridgeLib/Universal Bridge  Arms=1  SnubberResistance=1e6  SnubberCapacitance=inf  Device=IGBT / Diodes  Ron=1e-3  Lon=0  ForwardVoltages="[  1  1  ]"  ForwardVoltage=0  GTOparameters=[ 10e-6 , 20e-6 ]  IGBTparameters=[ 1e-6 , 2e-6 ]  Measurements=None  Measurements_2=None  converterType=Rectifier
  Vm1 : spsVoltageMeasurementLib/Voltage Measurement  PhasorSimulation=off  OutputType=Complex  PSBequivalent=0
  Vm3 : spsVoltageMeasurementLib/Voltage Measurement  PhasorSimulation=off  OutputType=Complex  PSBequivalent=0
  A : PMIOPort  Side=Left
  B : PMIOPort  Port=2  Side=Left
  Udc : Outport
  wires:
  Mux/1 -> Udc/1
  DRV/1 -> Demux3/1
  Demux3/2 -> Universal Bridge2/1
  Vm1/1 -> Mux/1
  Vm3/1 -> Mux/2
  Demux3/1 -> Universal Bridge1/1
  connections:
  Vm1/LConn2 -- C0/RConn1 -- Universal Bridge1/RConn2 -- Universal Bridge2/LConn1
  Universal Bridge1/LConn1 -- A/RConn1
  Vm3/LConn1 -- C1/LConn1 -- Universal Bridge2/RConn1
  Vm1/LConn1 -- Universal Bridge1/RConn1 -- C0/LConn1
  Universal Bridge2/RConn2 -- C1/RConn1 -- B/RConn1 -- Vm3/LConn2

== system MMC_21_Level_Rectifier/三电平级联混合MMC/Subsystem3/Subsystem/混合三电平子模块1 ==
  DRV : Inport
  C0 : spsSeriesRLCBranchLib/Series RLC Branch  LConnTagsString=__new0  RConnTagsString=__new0  BranchType=C  Resistance=0.1  Inductance=0  SetiL0=off  InitialCurrent=0  Capacitance=2e-3  Setx0=on  InitialVoltage=2200  Measurements=None
  C1 : spsSeriesRLCBranchLib/Series RLC Branch  LConnTagsString=__new0  RConnTagsString=__new0  BranchType=C  Resistance=0.1  Inductance=0  SetiL0=off  InitialCurrent=0  Capacitance=2e-3  Setx0=on  InitialVoltage=2200  Measurements=None
  Demux3 : Demux  Outputs=2
  Mux : Mux  Inputs=2
  Universal Bridge1 : spsUniversalBridgeLib/Universal Bridge  Arms=1  SnubberResistance=1e6  SnubberCapacitance=inf  Device=IGBT / Diodes  Ron=1e-3  Lon=0  ForwardVoltages="[  1  1  ]"  ForwardVoltage=0  GTOparameters=[ 10e-6 , 20e-6 ]  IGBTparameters=[ 1e-6 , 2e-6 ]  Measurements=None  Measurements_2=None  converterType=Rectifier
  Universal Bridge2 : spsUniversalBridgeLib/Universal Bridge  Arms=1  SnubberResistance=1e6  SnubberCapacitance=inf  Device=IGBT / Diodes  Ron=1e-3  Lon=0  ForwardVoltages="[  1  1  ]"  ForwardVoltage=0  GTOparameters=[ 10e-6 , 20e-6 ]  IGBTparameters=[ 1e-6 , 2e-6 ]  Measurements=None  Measurements_2=None  converterType=Rectifier
  Vm1 : spsVoltageMeasurementLib/Voltage Measurement  PhasorSimulation=off  OutputType=Complex  PSBequivalent=0
  Vm3 : spsVoltageMeasurementLib/Voltage Measurement  PhasorSimulation=off  OutputType=Complex  PSBequivalent=0
  A : PMIOPort  Side=Left
  B : PMIOPort  Port=2  Side=Left
  Udc : Outport
  wires:
  Demux3/1 -> Universal Bridge1/1
  Vm3/1 -> Mux/2
  Vm1/1 -> Mux/1
  Demux3/2 -> Universal Bridge2/1
  DRV/1 -> Demux3/1
  Mux/1 -> Udc/1
  connections:
  Vm3/LConn2 -- B/RConn1 -- C1/RConn1 -- Universal Bridge2/RConn2
  C0/LConn1 -- Universal Bridge1/RConn1 -- Vm1/LConn1
  Universal Bridge2/RConn1 -- C1/LConn1 -- Vm3/LConn1
  Universal Bridge1/LConn1 -- A/RConn1
  Universal Bridge2/LConn1 -- Universal Bridge1/RConn2 -- C0/RConn1 -- Vm1/LConn2

== system MMC_21_Level_Rectifier/三电平级联混合MMC/Subsystem3/Subsystem/混合三电平子模块2 ==
  DRV : Inport
  C0 : spsSeriesRLCBranchLib/Series RLC Branch  LConnTagsString=__new0  RConnTagsString=__new0  BranchType=C  Resistance=0.1  Inductance=0  SetiL0=off  InitialCurrent=0  Capacitance=2e-3  Setx0=on  InitialVoltage=2200  Measurements=None
  C1 : spsSeriesRLCBranchLib/Series RLC Branch  LConnTagsString=__new0  RConnTagsString=__new0  BranchType=C  Resistance=0.1  Inductance=0  SetiL0=off  InitialCurrent=0  Capacitance=2e-3  Setx0=on  InitialVoltage=2200  Measurements=None
  Demux3 : Demux  Outputs=2
  Mux : Mux  Inputs=2
  Universal Bridge1 : spsUniversalBridgeLib/Universal Bridge  Arms=1  SnubberResistance=1e6  SnubberCapacitance=inf  Device=IGBT / Diodes  Ron=1e-3  Lon=0  ForwardVoltages="[  1  1  ]"  ForwardVoltage=0  GTOparameters=[ 10e-6 , 20e-6 ]  IGBTparameters=[ 1e-6 , 2e-6 ]  Measurements=None  Measurements_2=None  converterType=Rectifier
  Universal Bridge2 : spsUniversalBridgeLib/Universal Bridge  Arms=1  SnubberResistance=1e6  SnubberCapacitance=inf  Device=IGBT / Diodes  Ron=1e-3  Lon=0  ForwardVoltages="[  1  1  ]"  ForwardVoltage=0  GTOparameters=[ 10e-6 , 20e-6 ]  IGBTparameters=[ 1e-6 , 2e-6 ]  Measurements=None  Measurements_2=None  converterType=Rectifier
  Vm1 : spsVoltageMeasurementLib/Voltage Measurement  PhasorSimulation=off  OutputType=Complex  PSBequivalent=0
  Vm3 : spsVoltageMeasurementLib/Voltage Measurement  PhasorSimulation=off  OutputType=Complex  PSBequivalent=0
  A : PMIOPort  Side=Left
  B : PMIOPort  Port=2  Side=Left
  Udc : Outport
  wires:
  Mux/1 -> Udc/1
  DRV/1 -> Demux3/1
  Demux3/2 -> Universal Bridge2/1
  Vm1/1 -> Mux/1
  Vm3/1 -> Mux/2
  Demux3/1 -> Universal Bridge1/1
  connections:
  Vm1/LConn2 -- C0/RConn1 -- Universal Bridge1/RConn2 -- Universal Bridge2/LConn1
  Universal Bridge1/LConn1 -- A/RConn1
  Vm3/LConn1 -- C1/LConn1 -- Universal Bridge2/RConn1
  Vm1/LConn1 -- Universal Bridge1/RConn1 -- C0/LConn1
  Universal Bridge2/RConn2 -- C1/RConn1 -- B/RConn1 -- Vm3/LConn2

== system MMC_21_Level_Rectifier/三电平级联混合MMC/Subsystem3/Subsystem/混合三电平子模块3 ==
  DRV : Inport
  C0 : spsSeriesRLCBranchLib/Series RLC Branch  LConnTagsString=__new0  RConnTagsString=__new0  BranchType=C  Resistance=0.1  Inductance=0  SetiL0=off  InitialCurrent=0  Capacitance=2e-3  Setx0=on  InitialVoltage=2200  Measurements=None
  C1 : spsSeriesRLCBranchLib/Series RLC Branch  LConnTagsString=__new0  RConnTagsString=__new0  BranchType=C  Resistance=0.1  Inductance=0  SetiL0=off  InitialCurrent=0  Capacitance=2e-3  Setx0=on  InitialVoltage=2200  Measurements=None
  Demux3 : Demux  Outputs=2
  Mux : Mux  Inputs=2
  Universal Bridge1 : spsUniversalBridgeLib/Universal Bridge  Arms=1  SnubberResistance=1e6  SnubberCapacitance=inf  Device=IGBT / Diodes  Ron=1e-3  Lon=0  ForwardVoltages="[  1  1  ]"  ForwardVoltage=0  GTOparameters=[ 10e-6 , 20e-6 ]  IGBTparameters=[ 1e-6 , 2e-6 ]  Measurements=None  Measurements_2=None  converterType=Rectifier
  Universal Bridge2 : spsUniversalBridgeLib/Universal Bridge  Arms=1  SnubberResistance=1e6  SnubberCapacitance=inf  Device=IGBT / Diodes  Ron=1e-3  Lon=0  ForwardVoltages="[  1  1  ]"  ForwardVoltage=0  GTOparameters=[ 10e-6 , 20e-6 ]  IGBTparameters=[ 1e-6 , 2e-6 ]  Measurements=None  Measurements_2=None  converterType=Rectifier
  Vm1 : spsVoltageMeasurementLib/Voltage Measurement  PhasorSimulation=off  OutputType=Complex  PSBequivalent=0
  Vm3 : spsVoltageMeasurementLib/Voltage Measurement  PhasorSimulation=off  OutputType=Complex  PSBequivalent=0
  A : PMIOPort  Side=Left
  B : PMIOPort  Port=2  Side=Left
  Udc : Outport
  wires:
  Demux3/1 -> Universal Bridge1/1
  Vm3/1 -> Mux/2
  Vm1/1 -> Mux/1
  Demux3/2 -> Universal Bridge2/1
  DRV/1 -> Demux3/1
  Mux/1 -> Udc/1
  connections:
  Vm3/LConn2 -- B/RConn1 -- C1/RConn1 -- Universal Bridge2/RConn2
  C0/LConn1 -- Universal Bridge1/RConn1 -- Vm1/LConn1
  Universal Bridge2/RConn1 -- C1/LConn1 -- Vm3/LConn1
  Universal Bridge1/LConn1 -- A/RConn1
  Universal Bridge2/LConn1 -- Universal Bridge1/RConn2 -- C0/RConn1 -- Vm1/LConn2

== system MMC_21_Level_Rectifier/三电平级联混合MMC/Subsystem3/Subsystem/混合三电平子模块4 ==
  DRV : Inport
  C0 : spsSeriesRLCBranchLib/Series RLC Branch  LConnTagsString=__new0  RConnTagsString=__new0  BranchType=C  Resistance=0.1  Inductance=0  SetiL0=off  InitialCurrent=0  Capacitance=2e-3  Setx0=on  InitialVoltage=2200  Measurements=None
  C1 : spsSeriesRLCBranchLib/Series RLC Branch  LConnTagsString=__new0  RConnTagsString=__new0  BranchType=C  Resistance=0.1  Inductance=0  SetiL0=off  InitialCurrent=0  Capacitance=2e-3  Setx0=on  InitialVoltage=2200  Measurements=None
  Demux3 : Demux  Outputs=2
  Mux : Mux  Inputs=2
  Universal Bridge1 : spsUniversalBridgeLib/Universal Bridge  Arms=1  SnubberResistance=1e6  SnubberCapacitance=inf  Device=IGBT / Diodes  Ron=1e-3  Lon=0  ForwardVoltages="[  1  1  ]"  ForwardVoltage=0  GTOparameters=[ 10e-6 , 20e-6 ]  IGBTparameters=[ 1e-6 , 2e-6 ]  Measurements=None  Measurements_2=None  converterType=Rectifier
  Universal Bridge2 : spsUniversalBridgeLib/Universal Bridge  Arms=1  SnubberResistance=1e6  SnubberCapacitance=inf  Device=IGBT / Diodes  Ron=1e-3  Lon=0  ForwardVoltages="[  1  1  ]"  ForwardVoltage=0  GTOparameters=[ 10e-6 , 20e-6 ]  IGBTparameters=[ 1e-6 , 2e-6 ]  Measurements=None  Measurements_2=None  converterType=Rectifier
  Vm1 : spsVoltageMeasurementLib/Voltage Measurement  PhasorSimulation=off  OutputType=Complex  PSBequivalent=0
  Vm3 : spsVoltageMeasurementLib/Voltage Measurement  PhasorSimulation=off  OutputType=Complex  PSBequivalent=0
  A : PMIOPort  Side=Left
  B : PMIOPort  Port=2  Side=Left
  Udc : Outport
  wires:
  Mux/1 -> Udc/1
  DRV/1 -> Demux3/1
  Demux3/2 -> Universal Bridge2/1
  Vm1/1 -> Mux/1
  Vm3/1 -> Mux/2
  Demux3/1 -> Universal Bridge1/1
  connections:
  Vm1/LConn2 -- C0/RConn1 -- Universal Bridge1/RConn2 -- Universal Bridge2/LConn1
  Universal Bridge1/LConn1 -- A/RConn1
  Vm3/LConn1 -- C1/LConn1 -- Universal Bridge2/RConn1
  Vm1/LConn1 -- Universal Bridge1/RConn1 -- C0/LConn1
  Universal Bridge2/RConn2 -- C1/RConn1 -- B/RConn1 -- Vm3/LConn2

== system MMC_21_Level_Rectifier/三电平级联混合MMC/Subsystem3/Subsystem/混合三电平子模块5 ==
  DRV : Inport
  C0 : spsSeriesRLCBranchLib/Series RLC Branch  LConnTagsString=__new0  RConnTagsString=__new0  BranchType=C  Resistance=0.1  Inductance=0  SetiL0=off  InitialCurrent=0  Capacitance=2e-3  Setx0=on  InitialVoltage=2200  Measurements=None
  C1 : spsSeriesRLCBranchLib/Series RLC Branch  LConnTagsString=__new0  RConnTagsString=__new0  BranchType=C  Resistance=0.1  Inductance=0  SetiL0=off  InitialCurrent=0  Capacitance=2e-3  Setx0=on  InitialVoltage=2200  Measurements=None
  Demux3 : Demux  Outputs=2
  Mux : Mux  Inputs=2
  Universal Bridge1 : spsUniversalBridgeLib/Universal Bridge  Arms=1  SnubberResistance=1e6  SnubberCapacitance=inf  Device=IGBT / Diodes  Ron=1e-3  Lon=0  ForwardVoltages="[  1  1  ]"  ForwardVoltage=0  GTOparameters=[ 10e-6 , 20e-6 ]  IGBTparameters=[ 1e-6 , 2e-6 ]  Measurements=None  Measurements_2=None  converterType=Rectifier
  Universal Bridge2 : spsUniversalBridgeLib/Universal Bridge  Arms=1  SnubberResistance=1e6  SnubberCapacitance=inf  Device=IGBT / Diodes  Ron=1e-3  Lon=0  ForwardVoltages="[  1  1  ]"  ForwardVoltage=0  GTOparameters=[ 10e-6 , 20e-6 ]  IGBTparameters=[ 1e-6 , 2e-6 ]  Measurements=None  Measurements_2=None  converterType=Rectifier
  Vm1 : spsVoltageMeasurementLib/Voltage Measurement  PhasorSimulation=off  OutputType=Complex  PSBequivalent=0
  Vm3 : spsVoltageMeasurementLib/Voltage Measurement  PhasorSimulation=off  OutputType=Complex  PSBequivalent=0
  A : PMIOPort  Side=Left
  B : PMIOPort  Port=2  Side=Left
  Udc : Outport
  wires:
  Demux3/1 -> Universal Bridge1/1
  Vm3/1 -> Mux/2
  Vm1/1 -> Mux/1
  Demux3/2 -> Universal Bridge2/1
  DRV/1 -> Demux3/1
  Mux/1 -> Udc/1
  connections:
  Vm3/LConn2 -- B/RConn1 -- C1/RConn1 -- Universal Bridge2/RConn2
  C0/LConn1 -- Universal Bridge1/RConn1 -- Vm1/LConn1
  Universal Bridge2/RConn1 -- C1/LConn1 -- Vm3/LConn1
  Universal Bridge1/LConn1 -- A/RConn1
  Universal Bridge2/LConn1 -- Universal Bridge1/RConn2 -- C0/RConn1 -- Vm1/LConn2

== system MMC_21_Level_Rectifier/三电平级联混合MMC/Subsystem3/Subsystem1/混合三电平子模块1 ==
  DRV : Inport
  C0 : spsSeriesRLCBranchLib/Series RLC Branch  LConnTagsString=__new0  RConnTagsString=__new0  BranchType=C  Resistance=0.1  Inductance=0  SetiL0=off  InitialCurrent=0  Capacitance=2e-3  Setx0=on  InitialVoltage=2200  Measurements=None
  C1 : spsSeriesRLCBranchLib/Series RLC Branch  LConnTagsString=__new0  RConnTagsString=__new0  BranchType=C  Resistance=0.1  Inductance=0  SetiL0=off  InitialCurrent=0  Capacitance=2e-3  Setx0=on  InitialVoltage=2200  Measurements=None
  Demux3 : Demux  Outputs=2
  Mux : Mux  Inputs=2
  Universal Bridge1 : spsUniversalBridgeLib/Universal Bridge  Arms=1  SnubberResistance=1e6  SnubberCapacitance=inf  Device=IGBT / Diodes  Ron=1e-3  Lon=0  ForwardVoltages="[  1  1  ]"  ForwardVoltage=0  GTOparameters=[ 10e-6 , 20e-6 ]  IGBTparameters=[ 1e-6 , 2e-6 ]  Measurements=None  Measurements_2=None  converterType=Rectifier
  Universal Bridge2 : spsUniversalBridgeLib/Universal Bridge  Arms=1  SnubberResistance=1e6  SnubberCapacitance=inf  Device=IGBT / Diodes  Ron=1e-3  Lon=0  ForwardVoltages="[  1  1  ]"  ForwardVoltage=0  GTOparameters=[ 10e-6 , 20e-6 ]  IGBTparameters=[ 1e-6 , 2e-6 ]  Measurements=None  Measurements_2=None  converterType=Rectifier
  Vm1 : spsVoltageMeasurementLib/Voltage Measurement  PhasorSimulation=off  OutputType=Complex  PSBequivalent=0
  Vm3 : spsVoltageMeasurementLib/Voltage Measurement  PhasorSimulation=off  OutputType=Complex  PSBequivalent=0
  A : PMIOPort  Side=Left
  B : PMIOPort  Port=2  Side=Left
  Udc : Outport
  wires:
  Mux/1 -> Udc/1
  DRV/1 -> Demux3/1
  Demux3/2 -> Universal Bridge2/1
  Vm1/1 -> Mux/1
  Vm3/1 -> Mux/2
  Demux3/1 -> Universal Bridge1/1
  connections:
  Vm1/LConn2 -- C0/RConn1 -- Universal Bridge1/RConn2 -- Universal Bridge2/LConn1
  Universal Bridge1/LConn1 -- A/RConn1
  Vm3/LConn1 -- C1/LConn1 -- Universal Bridge2/RConn1
  Vm1/LConn1 -- Universal Bridge1/RConn1 -- C0/LConn1
  Universal Bridge2/RConn2 -- C1/RConn1 -- B/RConn1 -- Vm3/LConn2

== system MMC_21_Level_Rectifier/三电平级联混合MMC/Subsystem3/Subsystem1/混合三电平子模块2 ==
  DRV : Inport
  C0 : spsSeriesRLCBranchLib/Series RLC Branch  LConnTagsString=__new0  RConnTagsString=__new0  BranchType=C  Resistance=0.1  Inductance=0  SetiL0=off  InitialCurrent=0  Capacitance=2e-3  Setx0=on  InitialVoltage=2200  Measurements=None
  C1 : spsSeriesRLCBranchLib/Series RLC Branch  LConnTagsString=__new0  RConnTagsString=__new0  BranchType=C  Resistance=0.1  Inductance=0  SetiL0=off  InitialCurrent=0  Capacitance=2e-3  Setx0=on  InitialVoltage=2200  Measurements=None
  Demux3 : Demux  Outputs=2
  Mux : Mux  Inputs=2
  Universal Bridge1 : spsUniversalBridgeLib/Universal Bridge  Arms=1  SnubberResistance=1e6  SnubberCapacitance=inf  Device=IGBT / Diodes  Ron=1e-3  Lon=0  ForwardVoltages="[  1  1  ]"  ForwardVoltage=0  GTOparameters=[ 10e-6 , 20e-6 ]  IGBTparameters=[ 1e-6 , 2e-6 ]  Measurements=None  Measurements_2=None  converterType=Rectifier
  Universal Bridge2 : spsUniversalBridgeLib/Universal Bridge  Arms=1  SnubberResistance=1e6  SnubberCapacitance=inf  Device=IGBT / Diodes  Ron=1e-3  Lon=0  ForwardVoltages="[  1  1  ]"  ForwardVoltage=0  GTOparameters=[ 10e-6 , 20e-6 ]  IGBTparameters=[ 1e-6 , 2e-6 ]  Measurements=None  Measurements_2=None  converterType=Rectifier
  Vm1 : spsVoltageMeasurementLib/Voltage Measurement  PhasorSimulation=off  OutputType=Complex  PSBequivalent=0
  Vm3 : spsVoltageMeasurementLib/Voltage Measurement  PhasorSimulation=off  OutputType=Complex  PSBequivalent=0
  A : PMIOPort  Side=Left
  B : PMIOPort  Port=2  Side=Left
  Udc : Outport
  wires:
  Demux3/1 -> Universal Bridge1/1
  Vm3/1 -> Mux/2
  Vm1/1 -> Mux/1
  Demux3/2 -> Universal Bridge2/1
  DRV/1 -> Demux3/1
  Mux/1 -> Udc/1
  connections:
  Vm3/LConn2 -- B/RConn1 -- C1/RConn1 -- Universal Bridge2/RConn2
  C0/LConn1 -- Universal Bridge1/RConn1 -- Vm1/LConn1
  Universal Bridge2/RConn1 -- C1/LConn1 -- Vm3/LConn1
  Universal Bridge1/LConn1 -- A/RConn1
  Universal Bridge2/LConn1 -- Universal Bridge1/RConn2 -- C0/RConn1 -- Vm1/LConn2

== system MMC_21_Level_Rectifier/三电平级联混合MMC/Subsystem3/Subsystem1/混合三电平子模块3 ==
  DRV : Inport
  C0 : spsSeriesRLCBranchLib/Series RLC Branch  LConnTagsString=__new0  RConnTagsString=__new0  BranchType=C  Resistance=0.1  Inductance=0  SetiL0=off  InitialCurrent=0  Capacitance=2e-3  Setx0=on  InitialVoltage=2200  Measurements=None
  C1 : spsSeriesRLCBranchLib/Series RLC Branch  LConnTagsString=__new0  RConnTagsString=__new0  BranchType=C  Resistance=0.1  Inductance=0  SetiL0=off  InitialCurrent=0  Capacitance=2e-3  Setx0=on  InitialVoltage=2200  Measurements=None
  Demux3 : Demux  Outputs=2
  Mux : Mux  Inputs=2
  Universal Bridge1 : spsUniversalBridgeLib/Universal Bridge  Arms=1  SnubberResistance=1e6  SnubberCapacitance=inf  Device=IGBT / Diodes  Ron=1e-3  Lon=0  ForwardVoltages="[  1  1  ]"  ForwardVoltage=0  GTOparameters=[ 10e-6 , 20e-6 ]  IGBTparameters=[ 1e-6 , 2e-6 ]  Measurements=None  Measurements_2=None  converterType=Rectifier
  Universal Bridge2 : spsUniversalBridgeLib/Universal Bridge  Arms=1  SnubberResistance=1e6  SnubberCapacitance=inf  Device=IGBT / Diodes  Ron=1e-3  Lon=0  ForwardVoltages="[  1  1  ]"  ForwardVoltage=0  GTOparameters=[ 10e-6 , 20e-6 ]  IGBTparameters=[ 1e-6 , 2e-6 ]  Measurements=None  Measurements_2=None  converterType=Rectifier
  Vm1 : spsVoltageMeasurementLib/Voltage Measurement  PhasorSimulation=off  OutputType=Complex  PSBequivalent=0
  Vm3 : spsVoltageMeasurementLib/Voltage Measurement  PhasorSimulation=off  OutputType=Complex  PSBequivalent=0
  A : PMIOPort  Side=Left
  B : PMIOPort  Port=2  Side=Left
  Udc : Outport
  wires:
  Mux/1 -> Udc/1
  DRV/1 -> Demux3/1
  Demux3/2 -> Universal Bridge2/1
  Vm1/1 -> Mux/1
  Vm3/1 -> Mux/2
  Demux3/1 -> Universal Bridge1/1
  connections:
  Vm1/LConn2 -- C0/RConn1 -- Universal Bridge1/RConn2 -- Universal Bridge2/LConn1
  Universal Bridge1/LConn1 -- A/RConn1
  Vm3/LConn1 -- C1/LConn1 -- Universal Bridge2/RConn1
  Vm1/LConn1 -- Universal Bridge1/RConn1 -- C0/LConn1
  Universal Bridge2/RConn2 -- C1/RConn1 -- B/RConn1 -- Vm3/LConn2
